simulink model "FCSMPC_double_vector_2025b"  (R2025b)
settings: Solver=FixedStepDiscrete  StartTime=0.0  StopTime=2  FixedStep=SimulinkTs  RelTol=1e-3
PreLoadFcn:
  | % Verzeichnis des Modells zum MATLAB-Pfad hinzufügen
  | modelDir = fileparts(get_param(bdroot, 'FileName'));
  | addpath(modelDir);
  | 
  | % Nur der Dateiname – kein Pfad!
  | set_param(bdroot, 'DataDictionary', 'FOC_params.sldd');
model workspace (MAT data in the model file):
  Np = Simulink.Parameter
  Np.Value = 5
  Np.Complexity = 'real'
  Np.Dimensions = [1 1]
  Np.DataType = 'double'
values from neighbouring files (symbols this model uses):
  Filter_Current_FilterTimeConst = 3.3333333333333335E-5    [FOC_params.sldd]
  Filter_Current_SensorTimeConst = 1.5915494309189535E-6    [FOC_params.sldd]
  FOC = evalin("base", "FOC")    [createFOC_SLDD.m]
  FOC_Control_Current_KIid = 10.0    [FOC_params.sldd]
  FOC_Control_Current_KIiq = 10.0    [FOC_params.sldd]
  FOC_Control_Current_KPid = 0.20418507462686566    [FOC_params.sldd]
  FOC_Control_Current_KPiq = 0.58674626865671642    [FOC_params.sldd]
  FOC_Control_Current_Krd = 0.8    [FOC_params.sldd]
  FOC_Control_Current_Krq = 0.8    [FOC_params.sldd]
  FOC_Control_Current_TclCur = 0.1    [FOC_params.sldd]
  FOC_Control_Current_Tnd = 0.1    [FOC_params.sldd]
  FOC_Control_Current_Tnq = 0.1    [FOC_params.sldd]
  FOC_Control_InverterVdc_V = 400.0    [FOC_params.sldd]
  FOC_Control_MotorImax_A = 650.0    [FOC_params.sldd]
  FOC_Control_MTPA_MTPV_nT_id_grid = -450.06704889786266 -439.56177000270145 -427.77784873303676 -416.66404703197372 -406.07553272717422 -395.15516533678584 -384.31176061747851 -374.03652088128132 -363.90551910193739 -353.79478643334204 -344.0221683092833 -334.51243453441936 -324.94614350292119 -315.21793409137081 -305.26543360965195 -295.21828280911944 -285.133916324101 -275.01232812136521 -264.86951532374729 -254.7797625148454 -244    [FOC_params.sldd]
  FOC_Control_MTPA_MTPV_nT_iq_grid = -449.09165648258488 -442.56958748923387 -437.25247759546528 -430.91792082419158 -423.83735797306491 -417.11730433547 -410.54064621830616 -403.71584331167304 -396.93611069310379 -390.15794305727007 -382.97216593027133 -375.44639668848538 -367.93447385667577 -360.57088856352266 -353.41289778449368 -346.34020584402072 -339.28416684923008 -332.22010880540631 -325.11927997033376 -317.92299905654966 -31    [FOC_params.sldd]
  FOC_Control_MTPA_MTPV_T_vec = -245.0 -240.0 -235.0 -230.0 -225.0 -220.0 -215.0 -210.0 -205.0 -200.0 -195.0 -190.0 -185.0 -180.0 -175.0 -170.0 -165.0 -160.0 -155.0 -150.0 -145.0 -140.0 -135.0 -130.0 -125.0 -120.0 -115.0 -110.0 -105.0 -100.0 -95.0 -90.0 -85.0 -80.0 -75.0 -70.0 -65.0 -60.0 -55.0 -50.0 -45.0 -40.0 -35.0 -30.0 -25.0 -20.0 -15.0 -10.0 -5.0 0.0 5.0 10.0 15.0 20.0 25.0 30.0 35.0 40.0 45.0 50.0 55.0 60.0 65.0 70.0 75.0    [FOC_params.sldd]
  FOC_Control_MTPA_MTPV_w_vec = 0.0 10.471975511965978 20.943951023931955 31.415926535897931 41.887902047863911 52.359877559829883 62.831853071795862 73.303828583761828 83.775804095727821 94.247779607693786 104.71975511965977 115.19173063162575 125.66370614359172 136.1356816555577 146.60765716752366 157.07963267948966 167.55160819145564 178.02358370342159 188.49555921538757 198.96753472735358 209.43951023931953 219.9114857512855    [FOC_params.sldd]
  FOC_Control_OpenLoop_Id_Ref_A = 0.0    [FOC_params.sldd]
  FOC_Control_OpenLoop_Iq_Ref_A = 0.0    [FOC_params.sldd]
  FOC_Control_OpenLoop_Ud_OpenLoop_V = 0.0    [FOC_params.sldd]
  FOC_Control_OpenLoop_Uq_OpenLoop_V = 0.0    [FOC_params.sldd]
  FOC_Control_RF_omegamech_rad_s = 3141.5926535897934    [FOC_params.sldd]
  FOC_Control_RF_RateCurrent_A = 500.0    [FOC_params.sldd]
  FOC_Control_RF_RateTrq_Nm = 500.0    [FOC_params.sldd]
  FOC_Control_theta_mechOffsetFix = 0.0    [FOC_params.sldd]
  FOC_Control_theta_mechOffsetTime = 0.0    [FOC_params.sldd]
  FOC_Control_TorqueRef_Nm = 10.0    [FOC_params.sldd]
  FOC_Control_Umax_V = 230.94010767585033    [FOC_params.sldd]
  FOC_Flag_ClosedLoopControl = 1.0    [FOC_params.sldd]
  FOC_Flag_ControlStrategy = 2.0    [FOC_params.sldd]
  FOC_Flag_PWMEnable = 1.0    [FOC_params.sldd]
  FOC_Flag_ResetControl = 0.0    [FOC_params.sldd]
  FOC_Flag_TorqueControl = 1.0    [FOC_params.sldd]
  FOC_LUT_DQLimiter_DQ_LUTScaling = 1.8749999999999995E-5    [FOC_params.sldd]
  FOC_PWM_AZSPWMMethod = 3.0    [FOC_params.sldd]
  FOC_PWM_HybridMode = 1.0    [FOC_params.sldd]
  FOC_PWM_LB1 = 0.5    [FOC_params.sldd]
  FOC_PWM_LB2 = 0.77    [FOC_params.sldd]
  FOC_PWM_PWMManuel = 1.0    [FOC_params.sldd]
  FOC_PWM_RSPWMMethod = 2.0    [FOC_params.sldd]
  FOC_PWM_UB1 = 0.66    [FOC_params.sldd]
  FOC_PWM_UB2 = 0.9    [FOC_params.sldd]
  FOC_SampleTime_TsCur = 0.0001    [FOC_params.sldd]
undefined symbols (not defined in the file or in its folder): dspblkCoreblockFVToolHelper, FCS, Filter, gcbh, Plant, SimulinkTs
libraries: hdlsllib x2, simulink x2, autolibfluxpmsm x1
(part 1 of 8)
settings Model: DataDictionary=FOC_params.sldd  Creator=kara  LastModifiedBy=Cheng
settings OptimizationCC: DefaultParameterBehavior=Inlined
settings DebuggingCC: ParameterPrecisionLossMsg=none
settings RTWCC: GPUComputeCapability=3.5

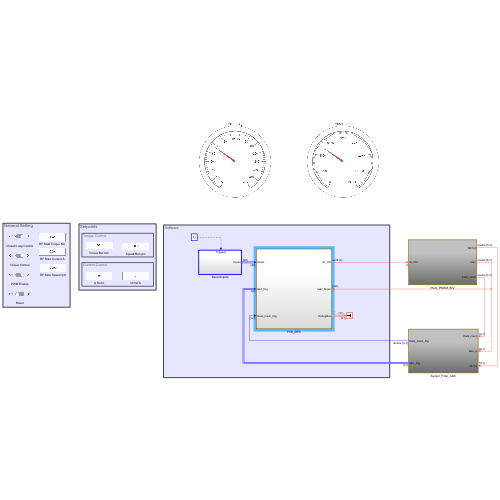
[thumbnail: Simulink's stored preview of the top-level diagram]
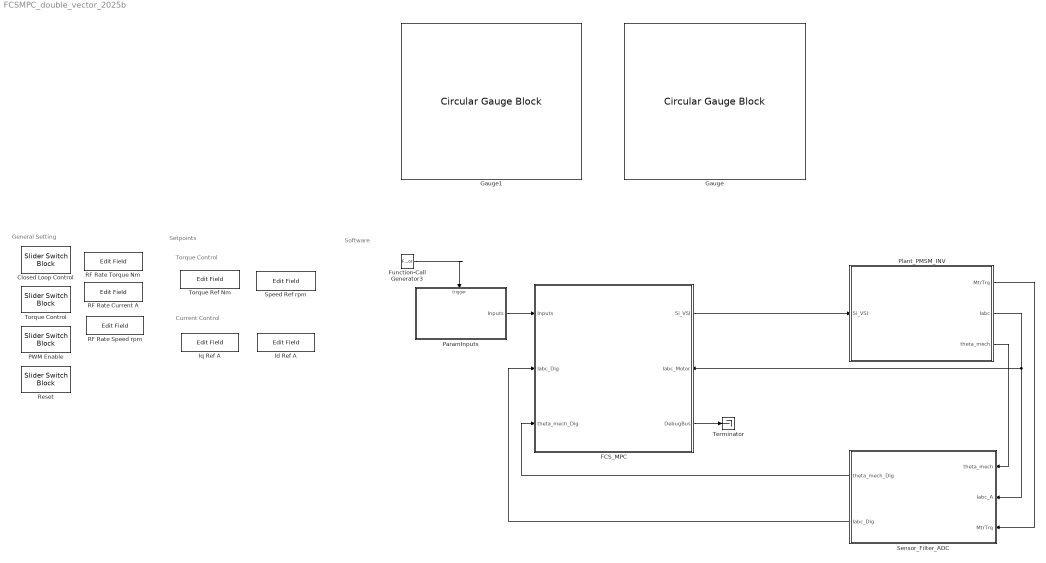
== system FCSMPC_double_vector_2025b ==
  note: Torque Control
  note: Software
  note: Current Control
  note: Setpoints
  note: General Setting
  Closed Loop Control : SliderSwitchBlock  LabelPosition=Hide
  FCS_MPC : Subsystem  VariantControl=AltPWM == 0
      settings: PortSchema="{\"entries\":[{\"content\":{\"sides\":[{\"content\":{\"connectorIds\":[\"In1\",\"In2\",\"In3\"]},\"type\":\"ConnectorPlacement.EquallySpacedRectSide\",\"uuid\":\"afdde33e-e0f4-4c11-9f6e-9de270b36af1\"},{\"content\":{\"connectorIds\":[\"Out1\",\"In4\",\"Out2\"],\"side\":\"RIGHT\"},\"type\":\"ConnectorPlacement.EquallySpacedRectSide\",\"uuid\":\"dc457a92-3b15-47da-9f19-4b6cbe74df3c\"},{\"content\":{\"side\":\"TOP\"},\"type\":\"ConnectorPlacement.EquallySpacedRectSide\",\"uuid\":\"233935a5-ca3c-43d9-bdde-90836d43fbe5\"}]},\"type\":\"ConnectorPlacement.EquallySpacedConnector\",\"uuid\":\"4f8af549-4a57-42d6-b429-a0a6155d0376\"}],\"packageUris\":[\"http://schema.mathworks.com/mf0/Connector/R2020b\"],\"version\":\"1.0\"}"
  Function-Call Generator3 : FunctionCallGenerator  SampleTime=FOC.SampleTime.TsSpeed
  Gauge : CircularGaugeBlock  ScaleMax=16000  FontColor=[0.0, 0.0, 0.0]
  Gauge1 : CircularGaugeBlock  ScaleMax=300  FontColor=[0.0, 0.0, 0.0]
  Id Ref A : EditField  LabelPosition=Hide  ShowInitialText=on  Alignment=Center
  Iq Ref A : EditField  LabelPosition=Hide  ShowInitialText=on  Alignment=Center
  PWM Enable : SliderSwitchBlock  LabelPosition=Hide
  ParamInputs : Subsystem
  Plant_PMSM_INV : Subsystem
  RF Rate Current A : EditField  LabelPosition=Hide  ShowInitialText=on  Alignment=Center
  RF Rate Speed rpm : EditField  LabelPosition=Hide  ShowInitialText=on  Alignment=Center
  RF Rate Torque Nm : EditField  LabelPosition=Hide  ShowInitialText=on  Alignment=Center
  Reset : SliderSwitchBlock  LabelPosition=Hide
  Sensor_Filter_ADC : Subsystem
  Speed Ref rpm : EditField  LabelPosition=Hide  ShowInitialText=on  Alignment=Center
  Terminator : Terminator
  Torque Control : SliderSwitchBlock  LabelPosition=Hide
  Torque Ref Nm : EditField  LabelPosition=Hide  ShowInitialText=on  Alignment=Center
  wires:
  ParamInputs/1(Inputs) -> FCS_MPC/1(Inputs)
  Function-Call Generator3/1 -> ParamInputs/Trigger
  Plant_PMSM_INV/2(Iabc) -> Sensor_Filter_ADC/2(Iabc_A), FCS_MPC/4(Iabc_Motor)
  Plant_PMSM_INV/3(theta_mech) -> Sensor_Filter_ADC/1(theta_mech)
  FCS_MPC/1(Si_VSI) -> Plant_PMSM_INV/1(Si_VSI)
  Sensor_Filter_ADC/1(theta_mech_Dig) -> FCS_MPC/3(theta_mech_Dig)
  Plant_PMSM_INV/1(MtrTrq) -> Sensor_Filter_ADC/3(MtrTrq)
  Sensor_Filter_ADC/2(Iabc_Dig) -> FCS_MPC/2(Iabc_Dig)
  FCS_MPC/2(DebugBus) -> Terminator/1

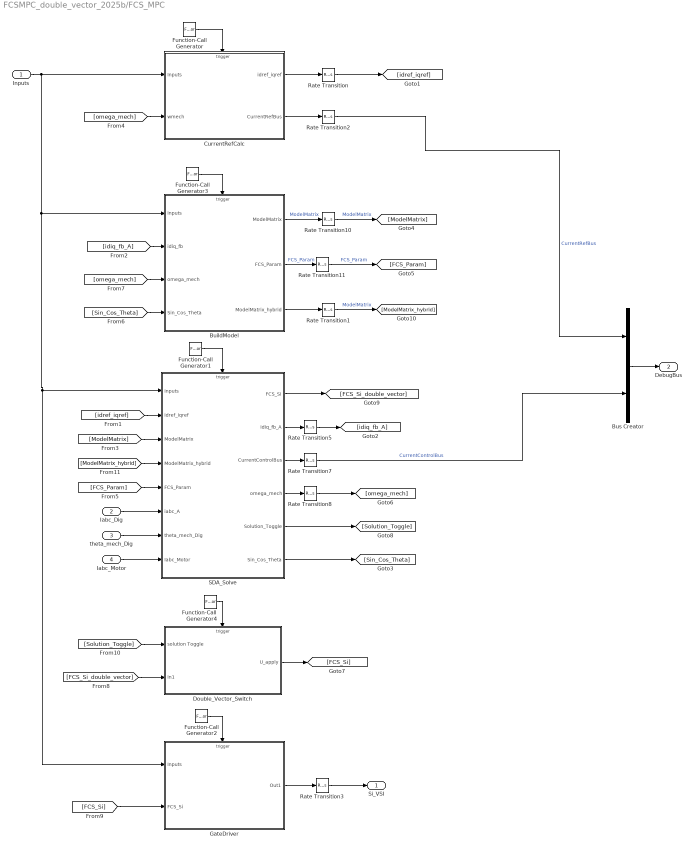
== system FCSMPC_double_vector_2025b/FCS_MPC ==
  Inputs : Inport
  Iabc_Dig : Inport  Port=2
  theta_mech_Dig : Inport  Port=3
  Iabc_Motor : Inport  Port=4
  BuildModel : Subsystem
  Bus Creator : BusCreator  Inputs=2
  CurrentRefCalc : Subsystem
  Double_Vector_Switch : Subsystem
  Function-Call Generator : FunctionCallGenerator  SampleTime=FOC.SampleTime.TsSpeed
  Function-Call Generator1 : FunctionCallGenerator  Priority=1  SampleTime=FCS.Ts_SDA
  Function-Call Generator2 : FunctionCallGenerator  Priority=3  SampleTime=FOC.SampleTime.BSW.DeadTimeSample
  Function-Call Generator3 : FunctionCallGenerator  SampleTime=FCS.Ts_BuildModel
  Function-Call Generator4 : FunctionCallGenerator  Priority=2  SampleTime=FCS.Ts_SDA/2
  GateDriver : Subsystem  TreatAsAtomicUnit=on
  Rate Transition{,1..3,5,7..8,10..11} (9 alike) : RateTransition  Deterministic=off
  SDA_Solve : Subsystem
  Si_VSI : Outport
  DebugBus : Outport  Port=2
  wires:
  Function-Call Generator/1 -> CurrentRefCalc/Trigger
  Function-Call Generator3/1 -> BuildModel/Trigger
  [omega_mech] -> CurrentRefCalc/2(wmech)
  CurrentRefCalc/1(idref_iqref) -> Rate Transition/1
  [idref_iqref] -> SDA_Solve/2(idref_iqref)
  Inputs/1 -> CurrentRefCalc/1(Inputs), GateDriver/1(Inputs), SDA_Solve/1(Inputs), BuildModel/1(Inputs)
  CurrentRefCalc/2(CurrentRefBus) -> Rate Transition2/1
  Bus Creator/1 -> DebugBus/1
  Rate Transition/1 -> [idref_iqref]
  Rate Transition2/1 -> Bus Creator/1  "CurrentRefBus"
  Rate Transition3/1 -> Si_VSI/1
  Function-Call Generator1/1 -> SDA_Solve/Trigger
  Iabc_Dig/1 -> SDA_Solve/6(iabc_A)
  SDA_Solve/2(idiq_fb_A) -> Rate Transition5/1
  Rate Transition5/1 -> [idiq_fb_A]
  [idiq_fb_A] -> BuildModel/2(idiq_fb)
  theta_mech_Dig/1 -> SDA_Solve/7(theta_mech_Dig)
  BuildModel/1(ModelMatrix) -> Rate Transition10/1  "ModelMatrix"
  BuildModel/2(FCS_Param) -> Rate Transition11/1  "FCS_Param"
  [ModelMatrix] -> SDA_Solve/3(ModelMatrix)
  [FCS_Param] -> SDA_Solve/5(FCS_Param)
  SDA_Solve/3(CurrentControlBus) -> Rate Transition7/1
  Rate Transition7/1 -> Bus Creator/2  "CurrentControlBus"
  SDA_Solve/4(omega_mech) -> Rate Transition8/1
  Rate Transition8/1 -> [omega_mech]
  [omega_mech] -> BuildModel/3(omega_mech)
  Rate Transition11/1 -> [FCS_Param]  "FCS_Param"
  Rate Transition10/1 -> [ModelMatrix]  "ModelMatrix"
  Function-Call Generator2/1 -> GateDriver/Trigger
  GateDriver/1(Out1) -> Rate Transition3/1
  [FCS_Si] -> GateDriver/2(FCS_Si)
  Function-Call Generator4/1 -> Double_Vector_Switch/Trigger
  [FCS_Si_double_vector] -> Double_Vector_Switch/2(In1)
  Double_Vector_Switch/1(U_apply) -> [FCS_Si]
  SDA_Solve/1(FCS_Si) -> [FCS_Si_double_vector]
  Iabc_Motor/1 -> SDA_Solve/8(Iabc_Motor)
  SDA_Solve/6(Sin_Cos_Theta) -> [Sin_Cos_Theta]
  [Sin_Cos_Theta] -> BuildModel/4(Sin_Cos_Theta)
  SDA_Solve/5(Solution_Toggle) -> [Solution_Toggle]
  [Solution_Toggle] -> Double_Vector_Switch/1(solution Toggle)
  BuildModel/3(ModelMatrix_hybrid) -> Rate Transition1/1
  Rate Transition1/1 -> [ModelMatrix_hybrid]  "ModelMatrix"
  [ModelMatrix_hybrid] -> SDA_Solve/4(ModelMatrix_hybrid)

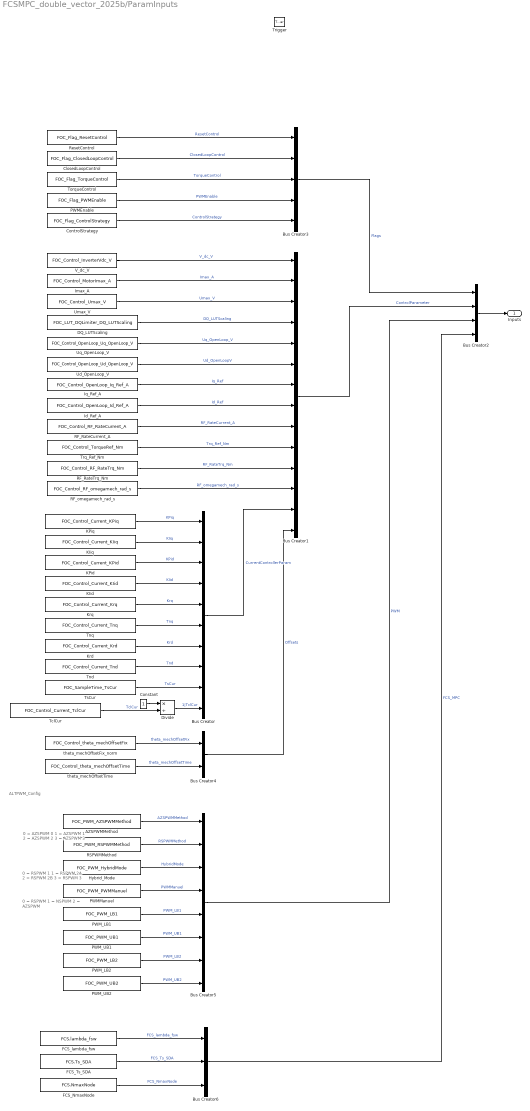
== system FCSMPC_double_vector_2025b/ParamInputs ==
  note: ALTPWM_Config
  note: 0 = RSPWM 1
      | 1 = RSPWM 2A
      | 2 = RSPWM 2B
      | 3 = RSPWM 3
  note: 0 = AZSPWM 0
      | 1 = AZSPWM 1
      | 2 = AZSPWM 2
      | 3 = AZSPWM 3
  note: 0 = RSPWM
      | 1 = NSPWM
      | 2 = AZSPWM
  Trigger : TriggerPort  TriggerType=function-call  VariantControl=(inherit)  SampleTimeType=periodic  SampleTime=FOC.SampleTime.TsSpeed  PortDimensions=1
  AZSPWMMethod : Constant  Value=FOC_PWM_AZSPWMMethod
  Bus Creator : BusCreator  Inputs=10
  Bus Creator1 : BusCreator  Inputs=14
  Bus Creator2 : BusCreator  Inputs=4
  Bus Creator3 : BusCreator  Inputs=5
  Bus Creator4 : BusCreator  Inputs=2
  Bus Creator5 : BusCreator  Inputs=8
  Bus Creator6 : BusCreator  Inputs=3
  ClosedLoopControl : Constant  Value=FOC_Flag_ClosedLoopControl
  Constant : Constant  OutDataTypeStr=SIScaling  SampleTime=-1
  ControlStrategy : Constant  Value=FOC_Flag_ControlStrategy
  DQ_LUTScaling : Constant  Value=FOC_LUT_DQLimiter_DQ_LUTScaling
  Divide : Product  Inputs=*/  OutDataTypeStr=SIScaling
  FCS_NmaxNode : Constant  Value=FCS.NmaxNode
  FCS_Ts_SDA : Constant  Value=FCS.Ts_SDA
  FCS_lambda_fsw : Constant  Value=FCS.lambda_fsw
  Hybrid_Mode : Constant  Value=FOC_PWM_HybridMode
  Id_Ref_A : Constant  Value=FOC_Control_OpenLoop_Id_Ref_A
  Imax_A : Constant  Value=FOC_Control_MotorImax_A
  Iq_Ref_A : Constant  Value=FOC_Control_OpenLoop_Iq_Ref_A
  KIid : Constant  Value=FOC_Control_Current_KIid
  KIiq : Constant  Value=FOC_Control_Current_KIiq
  KPid : Constant  Value=FOC_Control_Current_KPid
  KPiq : Constant  Value=FOC_Control_Current_KPiq
  Krd : Constant  Value=FOC_Control_Current_Krd
  Krq : Constant  Value=FOC_Control_Current_Krq
  PWMEnable : Constant  Value=FOC_Flag_PWMEnable
  PWMManuel : Constant  Value=FOC_PWM_PWMManuel
  PWM_LB1 : Constant  Value=FOC_PWM_LB1
  PWM_LB2 : Constant  Value=FOC_PWM_LB2
  PWM_UB1 : Constant  Value=FOC_PWM_UB1
  PWM_UB2 : Constant  Value=FOC_PWM_UB2
  RF_RateCurrent_A : Constant  Value=FOC_Control_RF_RateCurrent_A
  RF_RateTrq_Nm : Constant  Value=FOC_Control_RF_RateTrq_Nm
  RF_omegamech_rad_s : Constant  Value=FOC_Control_RF_omegamech_rad_s
  RSPWMMethod : Constant  Value=FOC_PWM_RSPWMMethod
  ResetControl : Constant  Value=FOC_Flag_ResetControl
  TclCur : Constant  Value=FOC_Control_Current_TclCur
  Tnd : Constant  Value=FOC_Control_Current_Tnd
  Tnq : Constant  Value=FOC_Control_Current_Tnq
  TorqueControl : Constant  Value=FOC_Flag_TorqueControl
  Trq_Ref_Nm : Constant  Value=FOC_Control_TorqueRef_Nm
  TsCur : Constant  Value=FOC_SampleTime_TsCur
  Ud_OpenLoop_V : Constant  Value=FOC_Control_OpenLoop_Ud_OpenLoop_V
  Umax_V : Constant  Value=FOC_Control_Umax_V
  Uq_OpenLoop_V : Constant  Value=FOC_Control_OpenLoop_Uq_OpenLoop_V
  V_dc_V : Constant  Value=FOC_Control_InverterVdc_V
  theta_mechOffsetFix_norm : Constant  Value=FOC_Control_theta_mechOffsetFix
  theta_mechOffsetTime : Constant  Value=FOC_Control_theta_mechOffsetTime
  Inputs : Outport
  wires:
  Bus Creator2/1 -> Inputs/1
  ClosedLoopControl/1 -> Bus Creator3/2  "ClosedLoopControl"
  TorqueControl/1 -> Bus Creator3/3  "TorqueControl"
  PWMEnable/1 -> Bus Creator3/4  "PWMEnable"
  Bus Creator3/1 -> Bus Creator2/1  "Flags"
  ResetControl/1 -> Bus Creator3/1  "ResetControl"
  ControlStrategy/1 -> Bus Creator3/5  "ControlStrategy"
  Ud_OpenLoop_V/1 -> Bus Creator1/6  "Ud_OpenLoopV"
  Uq_OpenLoop_V/1 -> Bus Creator1/5  "Uq_OpenLoop_V"
  DQ_LUTScaling/1 -> Bus Creator1/4  "DQ_LUTScaling"
  Umax_V/1 -> Bus Creator1/3  "Umax_V"
  Bus Creator1/1 -> Bus Creator2/2  "ControlParameter"
  Iq_Ref_A/1 -> Bus Creator1/7  "Iq_Ref"
  Id_Ref_A/1 -> Bus Creator1/8  "Id_Ref"
  Imax_A/1 -> Bus Creator1/2  "Imax_A"
  RF_RateTrq_Nm/1 -> Bus Creator1/11  "RF_RateTrq_Nm"
  Trq_Ref_Nm/1 -> Bus Creator1/10  "Trq_Ref_Nm"
  RF_RateCurrent_A/1 -> Bus Creator1/9  "RF_RateCurrent_A"
  Bus Creator/1 -> Bus Creator1/13  "CurrentControllerParam"
  V_dc_V/1 -> Bus Creator1/1  "V_dc_V"
  RF_omegamech_rad_s/1 -> Bus Creator1/12  "RF_omegamech_rad_s"
  theta_mechOffsetFix_norm/1 -> Bus Creator4/1  "theta_mechOffsetFix"
  theta_mechOffsetTime/1 -> Bus Creator4/2  "theta_mechOffsetTime"
  Bus Creator4/1 -> Bus Creator1/14  "Offsets"
  Bus Creator5/1 -> Bus Creator2/3  "PWM"
  PWM_UB1/1 -> Bus Creator5/6  "PWM_UB1"
  PWM_LB2/1 -> Bus Creator5/7  "PWM_LB2"
  AZSPWMMethod/1 -> Bus Creator5/1  "AZSPWMMethod"
  RSPWMMethod/1 -> Bus Creator5/2  "RSPWMMethod"
  PWM_LB1/1 -> Bus Creator5/5  "PWM_LB1"
  PWM_UB2/1 -> Bus Creator5/8  "PWM_UB2"
  Hybrid_Mode/1 -> Bus Creator5/3  "HybridMode"
  PWMManuel/1 -> Bus Creator5/4  "PWMManuel"
  TsCur/1 -> Bus Creator/9  "TsCur"
  KIiq/1 -> Bus Creator/2  "KIiq"
  Tnq/1 -> Bus Creator/6  "Tnq"
  Krd/1 -> Bus Creator/7  "Krd"
  KPid/1 -> Bus Creator/3  "KPid"
  Krq/1 -> Bus Creator/5  "Krq"
  Tnd/1 -> Bus Creator/8  "Tnd"
  KIid/1 -> Bus Creator/4  "KIid"
  KPiq/1 -> Bus Creator/1  "KPiq"
  TclCur/1 -> Divide/2  "TclCur"
  Divide/1 -> Bus Creator/10  "1|TclCur"
  Constant/1 -> Divide/1
  FCS_Ts_SDA/1 -> Bus Creator6/2  "FCS_Ts_SDA"
  FCS_lambda_fsw/1 -> Bus Creator6/1  "FCS_lambda_fsw"
  Bus Creator6/1 -> Bus Creator2/4  "FCS_MPC"
  FCS_NmaxNode/1 -> Bus Creator6/3  "FCS_NmaxNode"

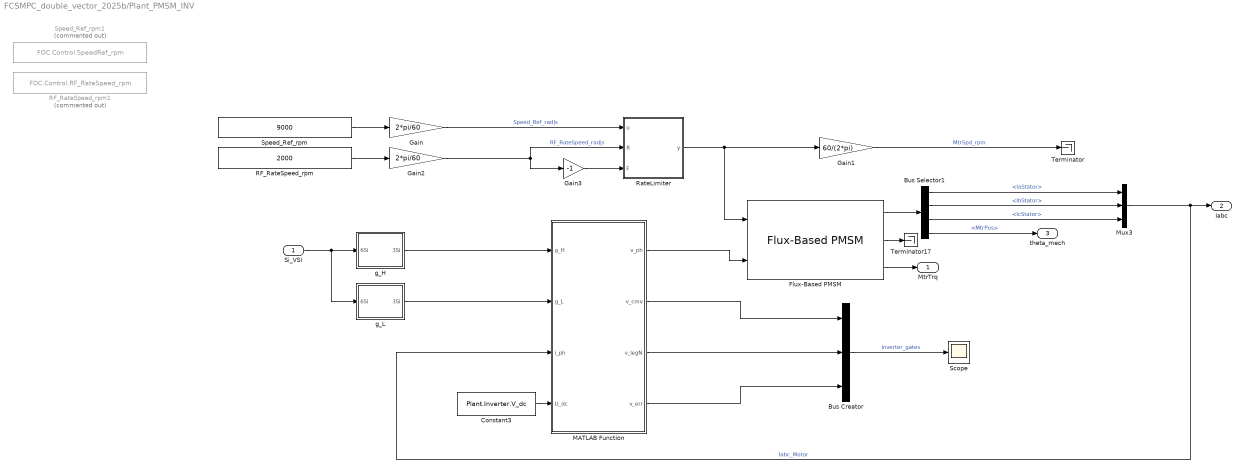
== system FCSMPC_double_vector_2025b/Plant_PMSM_INV ==
  Si_VSI : Inport
  Bus Creator : BusCreator  Inputs=3
  Bus Selector1 : BusSelector  OutputSignals=IaStator,IbStator,IcStator,MtrPos
  Constant3 : Constant  Value=Plant.Inverter.V_dc  SampleTime=-1
  Flux-Based PMSM : autolibfluxpmsm/Flux-Based PMSM  sim_type=Discrete  Ts=SimulinkTs  port_config=Speed  enable_hdl=off  flux_d=Plant.Fluxd_vec  n1=2  flux_q=Plant.Fluxq_vec  n2=2  id=Plant.FluxdFluxq_Id_grid'  iq=Plant.FluxdFluxq_Iq_grid'  preExtrapFlag=off  u1max=0.22457  u1min=-0.22607  u2max=0.42959  u2min=-0.4296  Rs=Plant.Motor.Rs  P=Plant.Motor.p  fluxdq0=[0 0]  theta_init=0  omega_init=0  mechanical=[0.0027, 4.924e-4, 0]  RefBlkName='autolibfluxpmsm/Flux-Based PMSM'  intPrec=23
      settings: LibrarySourceBlock=autolibemachines/Flux-Based PMSM
  Gain : Gain  Gain=2*pi/60
  Gain1 : Gain  Gain=60/(2*pi)
  Gain2 : Gain  Gain=2*pi/60
  Gain3 : Gain  Gain=-1
  MATLAB Function : MATLAB Function  TreatAsAtomicUnit=on
  Mux3 : Mux  Inputs=3
  RF_RateSpeed_rpm : Constant  Value=2000
  RF_RateSpeed_rpm1 : Constant  Commented=on  Value=FOC.Control.RF_RateSpeed_rpm
  RateLimiter : Stateflow chart  TreatAsAtomicUnit=on
  Scope : Scope
  Speed_Ref_rpm : Constant  Value=9000
  Speed_Ref_rpm1 : Constant  Commented=on  Value=FOC.Control.SpeedRef_rpm
  Terminator : Terminator
  Terminator17 : Terminator
  g_H : Subsystem
  g_L : Subsystem
  MtrTrq : Outport
  Iabc : Outport  Port=2
  theta_mech : Outport  Port=3
  wires:
  RateLimiter/1(y) -> Flux-Based PMSM/1, Gain1/1
  g_H/1(3Si) -> MATLAB Function/1(g_H)
  Bus Selector1/2 -> Mux3/2  "<IbStator>"
  Si_VSI/1 -> g_L/1(6Si), g_H/1(6Si)
  Bus Selector1/1 -> Mux3/1  "<IaStator>"
  Constant3/1 -> MATLAB Function/4(U_dc)
  Flux-Based PMSM/2 -> Terminator17/1
  Flux-Based PMSM/1 -> Bus Selector1/1
  Bus Selector1/3 -> Mux3/3  "<IcStator>"
  Gain1/1 -> Terminator/1  "MtrSpd_rpm"
  Flux-Based PMSM/3 -> MtrTrq/1
  Mux3/1 -> MATLAB Function/3(i_ph), Iabc/1  "Iabc_Motor"
  Bus Selector1/4 -> theta_mech/1  "<MtrPos>"
  Gain3/1 -> RateLimiter/3(F)
  RF_RateSpeed_rpm/1 -> Gain2/1
  Speed_Ref_rpm/1 -> Gain/1
  Gain/1 -> RateLimiter/1(u)  "Speed_Ref_rad|s"
  Gain2/1 -> RateLimiter/2(R), Gain3/1  "RF_RateSpeed_rad|s"
  g_L/1(3Si) -> MATLAB Function/2(g_L)
  MATLAB Function/1(v_ph) -> Flux-Based PMSM/2
  MATLAB Function/2(v_cmv) -> Bus Creator/1
  MATLAB Function/4(v_err) -> Bus Creator/3
  MATLAB Function/3(v_legN) -> Bus Creator/2
  Bus Creator/1 -> Scope/1  "inverter_gates"

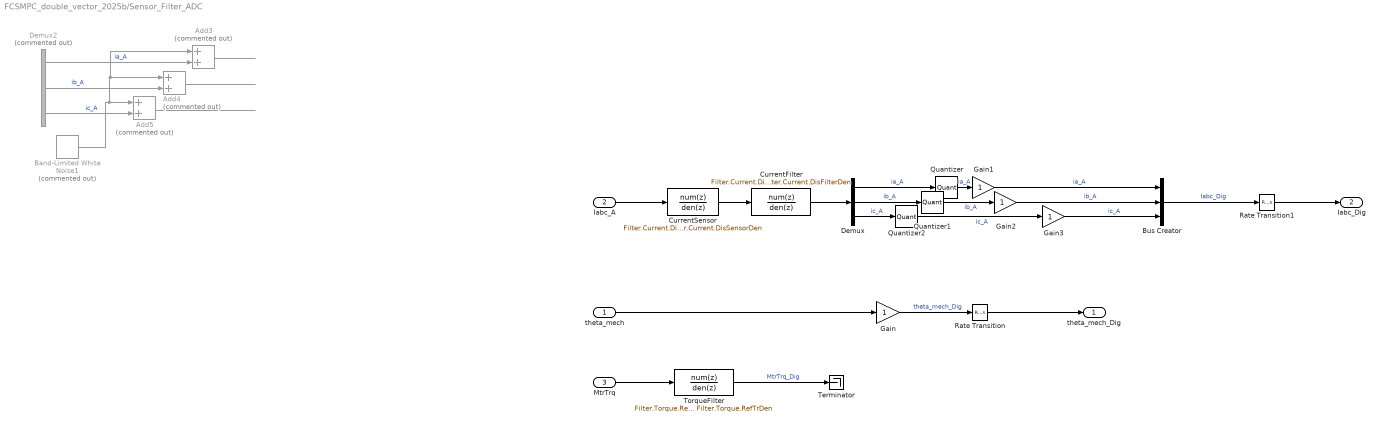
== system FCSMPC_double_vector_2025b/Sensor_Filter_ADC ==
  theta_mech : Inport
  Iabc_A : Inport  Port=2
  MtrTrq : Inport  Port=3
  Add3 : Sum  Commented=on
  Add4 : Sum  Commented=on
  Add5 : Sum  Commented=on
  Band-Limited White Noise1 : simulink/Sources/Band-Limited White Noise  Commented=on  Cov=[0.00001]  Ts=SimulinkTs  seed=[23341]
  Bus Creator : BusCreator  Inputs=3
  CurrentFilter : DiscreteTransferFcn  Numerator=Filter.Current.DisFilterNum  Denominator=Filter.Current.DisFilterDen
  CurrentSensor : DiscreteTransferFcn  LoadFcn=dspblkCoreblockFVToolHelper(gcbh,'load');  Numerator=Filter.Current.DisSensorNum  Denominator=Filter.Current.DisSensorDen
      settings: CopyFcn=dspblkCoreblockFVToolHelper(gcbh,'copy');  DeleteFcn=dspblkCoreblockFVToolHelper(gcbh,'close');  ModelCloseFcn=dspblkCoreblockFVToolHelper(gcbh,'close');  PreSaveFcn=dspblkCoreblockFVToolHelper(gcbh,'presave');  PostSaveFcn=dspblkCoreblockFVToolHelper(gcbh,'postsave');  CloseFcn=dspblkCoreblockFVToolHelper(gcbh,'close');
  Demux : Demux  Outputs=3
  Demux2 : Demux  Commented=on  Outputs=3
  Gain : Gain  OutDataTypeStr=HighScaling
  Gain1 : Gain  OutDataTypeStr=SIScaling
  Gain2 : Gain  OutDataTypeStr=SIScaling
  Gain3 : Gain  OutDataTypeStr=SIScaling
  Quantizer : Quantizer  QuantizationInterval=(10/32767)*264.04
  Quantizer1 : Quantizer  QuantizationInterval=(10/32767)*264.04
  Quantizer2 : Quantizer  QuantizationInterval=(10/32767)*264.04
  Rate Transition : RateTransition  Deterministic=off
  Rate Transition1 : RateTransition  Deterministic=off
  Terminator : Terminator
  TorqueFilter : DiscreteTransferFcn  Numerator=Filter.Torque.RefTrNum  Denominator=Filter.Torque.RefTrDen
  theta_mech_Dig : Outport
  Iabc_Dig : Outport  Port=2
  wires:
  MtrTrq/1 -> TorqueFilter/1
  CurrentSensor/1 -> CurrentFilter/1
  CurrentFilter/1 -> Demux/1
  TorqueFilter/1 -> Terminator/1  "MtrTrq_Dig"
  Demux/2 -> Quantizer1/1  "ib_A"
  Demux/3 -> Quantizer2/1  "ic_A"
  Demux/1 -> Quantizer/1  "ia_A"
  Bus Creator/1 -> Rate Transition1/1  "Iabc_Dig"
  Gain/1 -> Rate Transition/1  "theta_mech_Dig"
  Gain1/1 -> Bus Creator/1  "ia_A"
  Gain2/1 -> Bus Creator/2  "ib_A"
  Gain3/1 -> Bus Creator/3  "ic_A"
  Rate Transition/1 -> theta_mech_Dig/1
  Rate Transition1/1 -> Iabc_Dig/1
  theta_mech/1 -> Gain/1
  Quantizer/1 -> Gain1/1  "ia_A"
  Quantizer1/1 -> Gain2/1  "ib_A"
  Quantizer2/1 -> Gain3/1  "ic_A"
  Iabc_A/1 -> CurrentSensor/1
  Demux2/1 -> Add3/2  "ia_A"
  Demux2/2 -> Add4/2  "ib_A"
  Demux2/3 -> Add5/2  "ic_A"
  Add5/1 -> ?
  Add4/1 -> ?
  Add3/1 -> ?
  ? -> Demux2/1
  Band-Limited White Noise1/1 -> Add5/1, Add4/1, Add3/1

== system FCSMPC_double_vector_2025b/FCS_MPC/BuildModel ==
  Inputs : Inport
  idiq_fb : Inport  Port=2
  omega_mech : Inport  Port=3
  Sin_Cos_Theta : Inport  Port=4
  Trigger : TriggerPort  TriggerType=function-call  VariantControl=(inherit)  PropagateVarSize=Only when enabling  SampleTimeType=periodic  SampleTime=FCS.Ts_BuildModel  InitialTriggerSignalState=positive  PortDimensions=1
  BuildModel : Subsystem
  Bus Creator1 : BusCreator  Inputs=9
  Bus Selector : BusSelector  OutputSignals=FCS_MPC.FCS_Ts_SDA,ControlParameter.V_dc_V,FCS_MPC.FCS_lambda_fsw,FCS_MPC.FCS_NmaxNode
  Bus Selector1 : BusSelector  OutputSignals=Iq_fb_A,Id_fb_A
  Constant : Constant  Value=Plant.SimScapeTable.PM_const  OutDataTypeStr=PWMGenSacling  SampleTime=-1
  Constant1 : Constant  Value=Plant.Motor.Rs  OutDataTypeStr=PWMGenSacling  SampleTime=-1
  Gain : Gain  Gain=Plant.Motor.p  OutDataTypeStr=RoughScaling
  Ld_tab : Lookup_n-D  BreakpointsForDimension1=Plant.SimScapeTable.iQ_vec  BreakpointsForDimension2=Plant.SimScapeTable.iD_vec  Table=Plant.SimScapeTable.Ld_tab'  ExtrapMethod=Clip  InternalRulePriority=Speed  RndMeth=Simplest
      settings: InputPortMap=u0,u1
  Lq_tab : Lookup_n-D  BreakpointsForDimension1=Plant.SimScapeTable.iQ_vec  BreakpointsForDimension2=Plant.SimScapeTable.iD_vec  Table=Plant.SimScapeTable.Lq_tab'  ExtrapMethod=Clip  InternalRulePriority=Speed  RndMeth=Simplest
      settings: InputPortMap=u0,u1
  gain_double_switch1 : Gain  Gain=0.5
  ModelMatrix : Outport
  FCS_Param : Outport  Port=2
  ModelMatrix_hybrid : Outport  Port=3
  wires:
  Ld_tab/1 -> Bus Creator1/1  "Ld"
  Lq_tab/1 -> Bus Creator1/2  "Lq"
  Constant/1 -> Bus Creator1/4  "Psi"
  Bus Selector/2 -> Bus Creator1/7  "<V_dc_V>"
  Bus Creator1/1 -> FCS_Param/1, BuildModel/1(FCS_Param)
  BuildModel/1(ModelMatrix) -> ModelMatrix/1
  Bus Selector/4 -> Bus Creator1/9  "<FCS_NmaxNode>"
  Bus Selector/3 -> Bus Creator1/8  "<FCS_lambda_fsw>"
  idiq_fb/1 -> Bus Selector1/1
  Bus Selector1/2 -> Lq_tab/2, Ld_tab/2  "<Id_fb_A>"
  Bus Selector1/1 -> Lq_tab/1, Ld_tab/1  "<Iq_fb_A>"
  Constant1/1 -> Bus Creator1/3  "Rs"
  Inputs/1 -> Bus Selector/1
  Bus Selector/1 -> gain_double_switch1/1  "<FCS_Ts_SDA>"
  gain_double_switch1/1 -> Bus Creator1/6  "FCS_Ts_SDA_D_V"
  Gain/1 -> Bus Creator1/5  "wel"
  omega_mech/1 -> Gain/1
  Sin_Cos_Theta/1 -> BuildModel/2(Sin_Cos_Theta)
  BuildModel/2(ModelMatrix_hybrid) -> ModelMatrix_hybrid/1

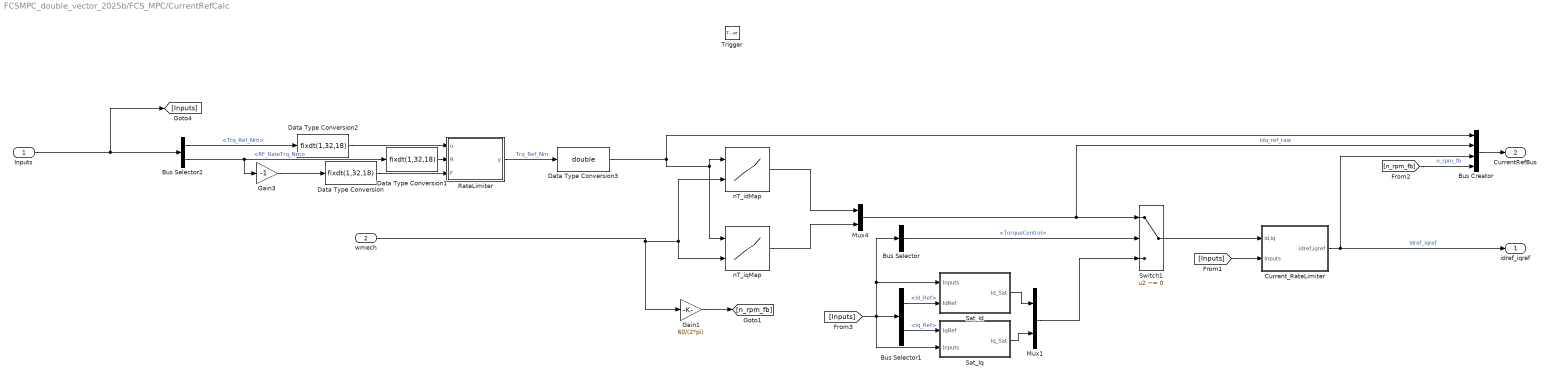
== system FCSMPC_double_vector_2025b/FCS_MPC/CurrentRefCalc ==
  Inputs : Inport
  wmech : Inport  Port=2
  Trigger : TriggerPort  TriggerType=function-call  VariantControl=(inherit)  PropagateVarSize=Only when enabling  SampleTimeType=periodic  SampleTime=FOC.SampleTime.TsSpeed  InitialTriggerSignalState=positive  PortDimensions=1
  Bus Creator : BusCreator  Inputs=4
  Bus Selector : BusSelector  OutputSignals=Flags.TorqueControl
  Bus Selector1 : BusSelector  OutputSignals=ControlParameter.Id_Ref,ControlParameter.Iq_Ref
  Bus Selector2 : BusSelector  OutputSignals=ControlParameter.Trq_Ref_Nm,ControlParameter.RF_RateTrq_Nm
  Current_RateLimiter : Subsystem
  Data Type Conversion : DataTypeConversion  OutDataTypeStr=fixdt(1,32,18)  SaturateOnIntegerOverflow=off  RndMeth=Floor
  Data Type Conversion1 : DataTypeConversion  OutDataTypeStr=fixdt(1,32,18)  SaturateOnIntegerOverflow=off  RndMeth=Floor
  Data Type Conversion2 : DataTypeConversion  OutDataTypeStr=fixdt(1,32,18)  SaturateOnIntegerOverflow=off  RndMeth=Floor
  Data Type Conversion3 : DataTypeConversion  OutDataTypeStr=double  SaturateOnIntegerOverflow=off  RndMeth=Floor
  Gain1 : Gain  Gain=60/(2*pi)  OutDataTypeStr=SIScaling
  Gain3 : Gain  Gain=-1  OutDataTypeStr=SIScaling
  Mux1 : Mux  Inputs=2
  Mux4 : Mux  Inputs=2
  RateLimiter : Stateflow chart  TreatAsAtomicUnit=on
  Sat_Id : Subsystem
  Sat_Iq : Subsystem
  Switch1 : Switch  Criteria=u2 ~= 0  OutDataTypeStr=SIScaling  SaturateOnIntegerOverflow=off  InputSameDT=off
  nT_idMap : Lookup_n-D  BreakpointsForDimension1=FOC_Control_MTPA_MTPV_T_vec  BreakpointsForDimension2=FOC_Control_MTPA_MTPV_w_vec  Table=FOC_Control_MTPA_MTPV_nT_id_grid  ExtrapMethod=Clip  InternalRulePriority=Speed  RndMeth=Simplest
      settings: InputPortMap=u0,u1
  nT_iqMap : Lookup_n-D  BreakpointsForDimension1=FOC_Control_MTPA_MTPV_T_vec  BreakpointsForDimension2=FOC_Control_MTPA_MTPV_w_vec  Table=FOC_Control_MTPA_MTPV_nT_iq_grid  ExtrapMethod=Clip  InternalRulePriority=Speed  RndMeth=Simplest
      settings: InputPortMap=u0,u1
  idref_iqref : Outport
  CurrentRefBus : Outport  Port=2
  wires:
  Bus Selector2/2 -> Data Type Conversion1/1, Gain3/1  "<RF_RateTrq_Nm>"
  Gain3/1 -> Data Type Conversion/1
  RateLimiter/1(y) -> Data Type Conversion3/1  "Trq_Ref_Nm"
  nT_iqMap/1 -> Mux4/2
  nT_idMap/1 -> Mux4/1
  Mux4/1 -> Bus Creator/2, Switch1/1  "idq_ref_raw"
  Bus Selector/1 -> Switch1/2  "<TorqueControl>"
  Bus Selector1/1 -> Sat_Id/2(IdRef)  "<Id_Ref>"
  Bus Selector1/2 -> Sat_Iq/1(IqRef)  "<Iq_Ref>"
  Mux1/1 -> Switch1/3
  Sat_Id/1(Id_Sat) -> Mux1/1
  Sat_Iq/1(Iq_Sat) -> Mux1/2
  Inputs/1 -> Bus Selector2/1, [Inputs]
  [Inputs] -> Sat_Iq/2(Inputs), Bus Selector/1, Sat_Id/1(Inputs), Bus Selector1/1
  Bus Selector2/1 -> Data Type Conversion2/1  "<Trq_Ref_Nm>"
  Switch1/1 -> Current_RateLimiter/1(id,iq)
  [Inputs] -> Current_RateLimiter/2(Inputs)
  Current_RateLimiter/1(idref,iqref) -> idref_iqref/1, Bus Creator/3  "idref_iqref"
  Bus Creator/1 -> CurrentRefBus/1
  [n_rpm_fb] -> Bus Creator/4  "n_rpm_fb"
  wmech/1 -> Gain1/1, nT_iqMap/2, nT_idMap/2
  Gain1/1 -> [n_rpm_fb]
  Data Type Conversion/1 -> RateLimiter/3(F)
  Data Type Conversion1/1 -> RateLimiter/2(R)
  Data Type Conversion2/1 -> RateLimiter/1(u)
  Data Type Conversion3/1 -> nT_iqMap/1, nT_idMap/1, Bus Creator/1

== system FCSMPC_double_vector_2025b/FCS_MPC/Double_Vector_Switch ==
  solution Toggle : Inport
  In1 : Inport  Port=2
  Trigger : TriggerPort  TriggerType=function-call  VariantControl=(inherit)  SampleTimeType=periodic  SampleTime=FCS.Ts_SDA/2  PortDimensions=1
  Demux : Demux  Outputs=2
  MATLAB Function : MATLAB Function  TreatAsAtomicUnit=on
  Terminator : Terminator
  Terminator1 : Terminator
  U_apply : Outport
  wires:
  In1/1 -> Demux/1
  Demux/1 -> MATLAB Function/1(UapplyFirst)
  Demux/2 -> MATLAB Function/2(UapplySecond)
  MATLAB Function/1(U_apply) -> U_apply/1  "U_apply"
  solution Toggle/1 -> MATLAB Function/3(solutionToggle)
  MATLAB Function/2(selectedHalf) -> Terminator/1  "selectedHalf"
  MATLAB Function/3(newSolutionDetected) -> Terminator1/1  "newSolutionDetected"

== system FCSMPC_double_vector_2025b/FCS_MPC/GateDriver ==
  Inputs : Inport
  FCS_Si : Inport  Port=2
  Trigger : TriggerPort  TriggerType=function-call  VariantControl=(inherit)  SampleTimeType=periodic  SampleTime=FOC.SampleTime.BSW.DeadTimeSample
  Bus Selector : BusSelector  OutputSignals=Flags.PWMEnable
  Constant4 : Constant  Value=[0 0 0 0 0 0]  OutDataTypeStr=uint8  SampleTime=-1
  GateDriver : Subsystem  ReferencedSubsystem=GateDriver  DeadTime=FOC.SampleTime.BSW.DeadTime  DeadTimeSample=FOC.SampleTime.BSW.DeadTimeSample
  Switch1 : Switch  Criteria=u2 ~= 0  SaturateOnIntegerOverflow=off  InputSameDT=off
  Out1 : Outport
  wires:
  GateDriver/1 -> Switch1/1
  Constant4/1 -> Switch1/3
  Switch1/1 -> Out1/1  "Si_VSI"
  Inputs/1 -> Bus Selector/1
  Bus Selector/1 -> Switch1/2  "<PWMEnable>"
  FCS_Si/1 -> GateDriver/1  "U_apply_Switch"

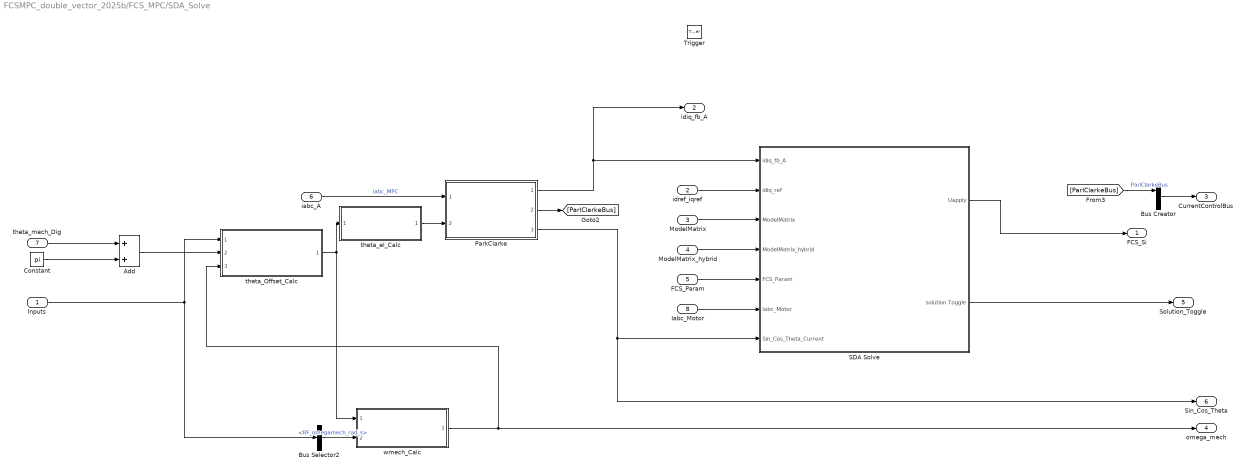
== system FCSMPC_double_vector_2025b/FCS_MPC/SDA_Solve ==
  Inputs : Inport
  idref_iqref : Inport  Port=2
  ModelMatrix : Inport  Port=3
  ModelMatrix_hybrid : Inport  Port=4
  FCS_Param : Inport  Port=5
  iabc_A : Inport  Port=6
  theta_mech_Dig : Inport  Port=7
  Iabc_Motor : Inport  Port=8
  Trigger : TriggerPort  TriggerType=function-call  VariantControl=(inherit)  PropagateVarSize=Only when enabling  SampleTimeType=periodic  SampleTime=FCS.Ts_SDA  InitialTriggerSignalState=positive  PortDimensions=1
  Add : Sum  OutDataTypeStr=HighScaling
  Bus Creator : BusCreator  Inputs=2
  Bus Selector2 : BusSelector  OutputSignals=ControlParameter.RF_omegamech_rad_s
  Constant : Constant  Value=pi  OutDataTypeStr=HighScaling
  ParkClarke : Subsystem  ReferencedSubsystem=ParkClarke
  SDA Solve : Subsystem  VariantControl=MPC_VARIANT == 2
  theta_Offset_Calc : Subsystem  ReferencedSubsystem=theta_Offset_Calc
  theta_el_Calc : Subsystem  ReferencedSubsystem=theta_el_Calc
  wmech_Calc : Subsystem  ReferencedSubsystem=wmech_Calc
  FCS_Si : Outport
  idiq_fb_A : Outport  Port=2
  CurrentControlBus : Outport  Port=3
  omega_mech : Outport  Port=4
  Solution_Toggle : Outport  Port=5
  Sin_Cos_Theta : Outport  Port=6
  wires:
  ParkClarke/1 -> SDA Solve/1(idiq_fb_A), idiq_fb_A/1
  wmech_Calc/1 -> omega_mech/1, theta_Offset_Calc/3
  theta_Offset_Calc/1 -> wmech_Calc/1, theta_el_Calc/1
  ParkClarke/2 -> [ParlClarkeBus]
  theta_el_Calc/1 -> ParkClarke/2
  iabc_A/1 -> ParkClarke/1  "iabc_MPC"
  Add/1 -> theta_Offset_Calc/2
  theta_mech_Dig/1 -> Add/1
  Constant/1 -> Add/2
  [ParlClarkeBus] -> Bus Creator/1  "ParlClarkeBus"
  Bus Creator/1 -> CurrentControlBus/1
  ParkClarke/3 -> Sin_Cos_Theta/1, SDA Solve/7(Sin_Cos_Theta_Current)
  idref_iqref/1 -> SDA Solve/2(idiq_ref)
  ModelMatrix/1 -> SDA Solve/3(ModelMatrix)
  FCS_Param/1 -> SDA Solve/5(FCS_Param)
  ? -> Bus Creator/2  "SDA Bus"
  SDA Solve/1(Uapply) -> FCS_Si/1
  Iabc_Motor/1 -> SDA Solve/6(Iabc_Motor)
  Inputs/1 -> Bus Selector2/1, theta_Offset_Calc/1
  Bus Selector2/1 -> wmech_Calc/2  "<RF_omegamech_rad_s>"
  SDA Solve/2(solution Toggle) -> Solution_Toggle/1
  ModelMatrix_hybrid/1 -> SDA Solve/4(ModelMatrix_hybrid)

== system FCSMPC_double_vector_2025b/Plant_PMSM_INV/g_H ==
  6Si : Inport
  Demux2 : Demux  Outputs=6
  Mux2 : Mux  Inputs=3
  Terminator12 : Terminator
  Terminator13 : Terminator
  Terminator14 : Terminator
  3Si : Outport
  wires:
  Demux2/1 -> Mux2/1
  Demux2/3 -> Mux2/2
  Demux2/2 -> Terminator12/1
  Demux2/4 -> Terminator13/1
  Demux2/5 -> Mux2/3
  Demux2/6 -> Terminator14/1
  Mux2/1 -> 3Si/1
  6Si/1 -> Demux2/1

== system FCSMPC_double_vector_2025b/Plant_PMSM_INV/g_L ==
  6Si : Inport
  Demux2 : Demux  Outputs=6
  Mux2 : Mux  Inputs=3
  Terminator1 : Terminator
  Terminator13 : Terminator
  Terminator14 : Terminator
  3Si : Outport
  wires:
  6Si/1 -> Demux2/1
  Mux2/1 -> 3Si/1
  Demux2/6 -> Mux2/3
  Demux2/5 -> Terminator14/1
  Demux2/4 -> Mux2/2
  Demux2/2 -> Mux2/1
  Demux2/3 -> Terminator13/1
  Demux2/1 -> Terminator1/1
